simulink model "TEC_Electrothermal_ClosedLoop"  (R2022b)
settings: Solver=ode15s  StartTime=0.0  StopTime=2400  MaxStep=1  RelTol=1e-6  AbsTol=1e-8
model workspace (MAT data in the model file):
  TEC_parameters = [24 0.8 0.012578468121 0.070126334619 4.5 0.02 3 3.6 0.25 0.012 0.2 500]
  switching_mode = 0
libraries: fl_lib x11, nesl_utility x5, ee_lib x1
settings Model: Creator=Greatlovers  LastModifiedBy=Greatlovers

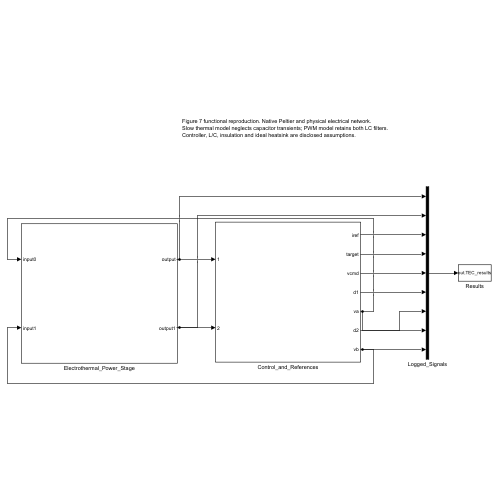
[thumbnail: Simulink's stored preview of the top-level diagram]
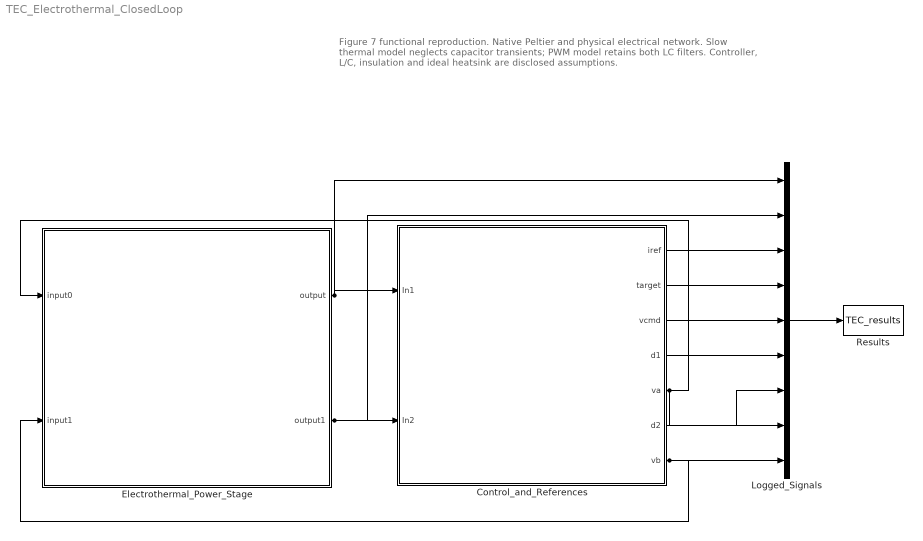
== system TEC_Electrothermal_ClosedLoop ==
  note: Figure 7 functional reproduction. Native Peltier and physical electrical network.
      | Slow thermal model neglects capacitor transients; PWM model retains both LC filters.
      | Controller, L/C, insulation and ideal heatsink are disclosed assumptions.
  Control_and_References : Subsystem
  Electrothermal_Power_Stage : Subsystem
  Logged_Signals : Mux  Inputs=9
  Results : ToWorkspace  VariableName=TEC_results  SaveFormat=Timeseries  SampleTime=-1
  wires:
  Control_and_References/4(d1) -> Logged_Signals/6
  Electrothermal_Power_Stage/1(output) -> Logged_Signals/1, Control_and_References/1(In1)
  Control_and_References/3(vcmd) -> Logged_Signals/5
  Control_and_References/1(iref) -> Logged_Signals/3
  Electrothermal_Power_Stage/2(output1) -> Logged_Signals/2, Control_and_References/2(In2)
  Control_and_References/2(target) -> Logged_Signals/4
  Control_and_References/5(va) -> Electrothermal_Power_Stage/1(input0), Logged_Signals/8
  Control_and_References/6(d2) -> Logged_Signals/7
  Control_and_References/7(vb) -> Electrothermal_Power_Stage/2(input1), Logged_Signals/9
  Logged_Signals/1 -> Results/1

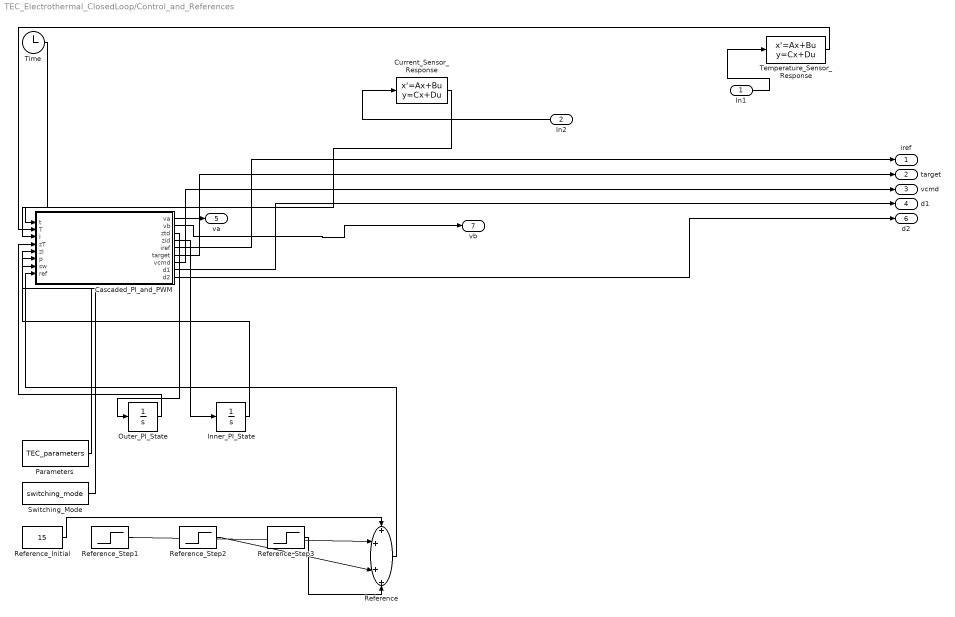
== system TEC_Electrothermal_ClosedLoop/Control_and_References ==
  In1 : Inport
  In2 : Inport  Port=2
  Cascaded_PI_and_PWM : MATLAB Function  TreatAsAtomicUnit=on
  Current_Sensor_Response : StateSpace  A=-1e5  B=1e5  D=0  InitialCondition=0
  Inner_PI_State : Integrator
  Outer_PI_State : Integrator
  Parameters : Constant  Value=TEC_parameters
  Reference : Sum  Inputs=++++
  Reference_Initial : Constant  Value=15
  Reference_Step1 : Step  Time=600  After=40  SampleTime=0
  Reference_Step2 : Step  Time=1200  After=-70  SampleTime=0
  Reference_Step3 : Step  Time=1800  After=110  SampleTime=0
  Switching_Mode : Constant  Value=switching_mode
  Temperature_Sensor_Response : StateSpace  A=-100  B=100  D=0  InitialCondition=298.15
  Time : Clock
  iref : Outport
  target : Outport  Port=2
  vcmd : Outport  Port=3
  d1 : Outport  Port=4
  va : Outport  Port=5
  d2 : Outport  Port=6
  vb : Outport  Port=7
  wires:
  Reference_Step3/1 -> Reference/4
  Reference_Initial/1 -> Reference/1
  Outer_PI_State/1 -> Cascaded_PI_and_PWM/4(zT)
  Cascaded_PI_and_PWM/1(va) -> va/1
  Time/1 -> Cascaded_PI_and_PWM/1(t)
  Reference_Step1/1 -> Reference/2
  Current_Sensor_Response/1 -> Cascaded_PI_and_PWM/3(I)
  Switching_Mode/1 -> Cascaded_PI_and_PWM/7(sw)
  Cascaded_PI_and_PWM/9(d2) -> d2/1
  Reference/1 -> Cascaded_PI_and_PWM/8(ref)
  Temperature_Sensor_Response/1 -> Cascaded_PI_and_PWM/2(T)
  Reference_Step2/1 -> Reference/3
  Cascaded_PI_and_PWM/5(iref) -> iref/1
  Inner_PI_State/1 -> Cascaded_PI_and_PWM/5(zI)
  Parameters/1 -> Cascaded_PI_and_PWM/6(p)
  Cascaded_PI_and_PWM/3(ztd) -> Outer_PI_State/1
  In1/1 -> Temperature_Sensor_Response/1
  Cascaded_PI_and_PWM/4(zid) -> Inner_PI_State/1
  In2/1 -> Current_Sensor_Response/1
  Cascaded_PI_and_PWM/8(d1) -> d1/1
  Cascaded_PI_and_PWM/2(vb) -> vb/1
  Cascaded_PI_and_PWM/7(vcmd) -> vcmd/1
  Cascaded_PI_and_PWM/6(target) -> target/1

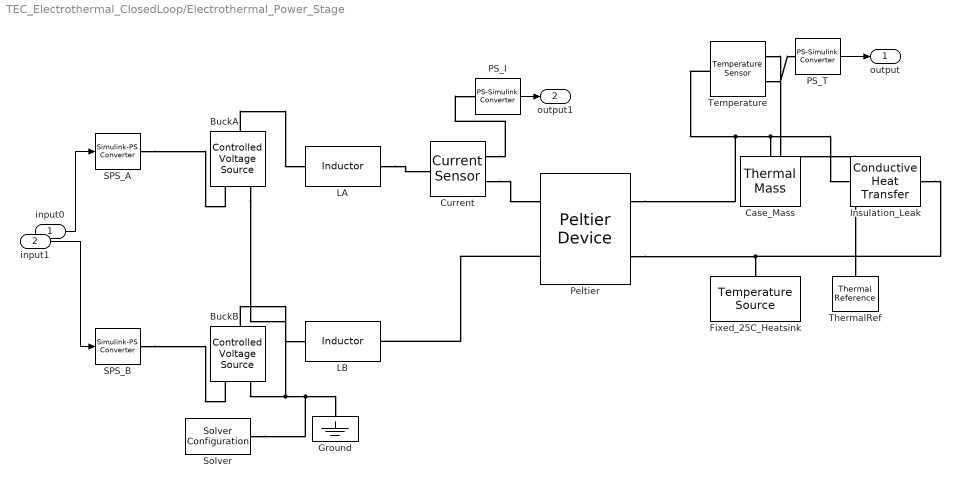
== system TEC_Electrothermal_ClosedLoop/Electrothermal_Power_Stage ==
  input0 : Inport
  input1 : Inport  Port=2
  BuckA : fl_lib/Electrical/Electrical Sources/Controlled Voltage Source
  BuckB : fl_lib/Electrical/Electrical Sources/Controlled Voltage Source
  Case_Mass : fl_lib/Thermal/Thermal Elements/Thermal Mass  mass=0.005 kg  sp_heat=900 J/(K*kg)  num_ports=foundation.enum.numPorts2.one  T_specify=on  T_priority=High  T=298.15 K  T_nominal_specify=off  T_nominal_unit=K  T_nominal_value=1  Q_specify=off  Q_priority=None  Q=0 W  Q_nominal_specify=off  Q_nominal_unit=W  Q_nominal_value=1
  Current : fl_lib/Electrical/Electrical Sensors/Current Sensor
  Fixed_25C_Heatsink : fl_lib/Thermal/Thermal Sources/Temperature Source  temperature=298.15 K
  Ground : fl_lib/Electrical/Electrical Elements/Electrical Reference
  Insulation_Leak : fl_lib/Thermal/Thermal Elements/Conductive Heat Transfer  thermal_type=foundation.enum.ConstantVariableTabulated.Constant  wall_geometry=foundation.enum.ConductionWallGeometry.Planar  area=0.001 m^2  thickness=0.05 m  d_in=0.05 m  d_out=0.1 m  L=1 m  th_cond_min=10 W/(K*m)  th_cond=1 W/(K*m)  th_cond_TLU=[413, 401, 392, 383, 371, 357, 342] W/(K*m)  temp_TLU=[200, 273, 400, 600, 800, 1000, 1200] K  T_specify=off  T_priority=None  T=0 K  T_nominal_specify=off  T_nominal_unit=K  T_nominal_value=1  Q_specify=off  Q_priority=None  Q=0 W  Q_nominal_specify=off  Q_nominal_unit=W  Q_nominal_value=1
  LA : fl_lib/Electrical/Electrical Elements/Inductor  l=220e-6 H  r=0.03 Ohm  g=1e-9 1/Ohm  i_specify=off  i_priority=None  i=0 A  i_nominal_specify=off  i_nominal_unit=A  i_nominal_value=1  v_specify=off  v_priority=None  v=0 V  v_nominal_specify=off  v_nominal_unit=V  v_nominal_value=1  i_L_specify=off  i_L_priority=High  i_L=0 A  i_L_nominal_specify=off  i_L_nominal_unit=A  i_L_nominal_value=1
  LB : fl_lib/Electrical/Electrical Elements/Inductor  l=220e-6 H  r=0.03 Ohm  g=1e-9 1/Ohm  i_specify=off  i_priority=None  i=0 A  i_nominal_specify=off  i_nominal_unit=A  i_nominal_value=1  v_specify=off  v_priority=None  v=0 V  v_nominal_specify=off  v_nominal_unit=V  v_nominal_value=1  i_L_specify=off  i_L_priority=High  i_L=0 A  i_L_nominal_specify=off  i_L_nominal_unit=A  i_L_nominal_value=1
  PS_I : nesl_utility/PS-Simulink Converter  PhysicalDomain=network_engine_domain  SubClassName=ps_output  LeftPortType=input  RightPortType=output  PseudoPeriodic=off  Frequencies=[]  VectorFormat=inherit  Unit=A  AffineConversion=off
  PS_T : nesl_utility/PS-Simulink Converter  PhysicalDomain=network_engine_domain  SubClassName=ps_output  LeftPortType=input  RightPortType=output  PseudoPeriodic=off  Frequencies=[]  VectorFormat=inherit  Unit=K  AffineConversion=off
  Peltier : ee_lib/Sensors & Transducers/Peltier Device  alpha=TEC_parameters(3) V/K  R=TEC_parameters(2) Ohm  K=TEC_parameters(4) W/K
      settings: InternalSimscapePortConfiguration="{\"Bottom\":[],\"Left\":[{\"id\":\"p\",\"label\":\"+\",\"type\":\"foundation.electrical.electrical\"},{\"id\":\"n\",\"label\":\"-\",\"type\":\"foundation.electrical.electrical\"}],\"Right\":[{\"id\":\"A\",\"label\":\"A\",\"type\":\"foundation.thermal.thermal\"},{\"id\":\"B\",\"label\":\"B\",\"type\":\"foundation.thermal.thermal\"}],\"Top\":[]}"
  SPS_A : nesl_utility/Simulink-PS Converter  PhysicalDomain=network_engine_domain  SubClassName=ps_input  LeftPortType=input  RightPortType=output  PseudoPeriodic=off  Frequencies=[]  NoiseDistribution=none  NoiseParameters=[]  Unit=V  AffineConversion=off  FilteringAndDerivatives=zero  SimscapeFilterOrder=1  InputFilterTimeConstant=0.001  UdotUserProvided=0
  SPS_B : nesl_utility/Simulink-PS Converter  PhysicalDomain=network_engine_domain  SubClassName=ps_input  LeftPortType=input  RightPortType=output  PseudoPeriodic=off  Frequencies=[]  NoiseDistribution=none  NoiseParameters=[]  Unit=V  AffineConversion=off  FilteringAndDerivatives=zero  SimscapeFilterOrder=1  InputFilterTimeConstant=0.001  UdotUserProvided=0
  Solver : nesl_utility/Solver Configuration  PhysicalDomain=network_engine_domain  SubClassName=solver  LeftPortType=input  RightPortType=generic  Tones=[]  Harmonics=[]  SimulateNoise=off  Profile=off  UseLocalSampling=off  EnableSwitchedLinearOptims=on  FrequencyDomain=off  UseCCode=off  RelTol=0.001  AbsTol=0.001  MinStep=1e-09  ToWorkspace=off  RevertToSquareIcSolve=off  NumHomotopyIterations=100  PhasorMode=off  PhasorModeNumHarmonics=1  ConsistencySolver=NEWTON_XTOL_AFTER_FTOL  IndexReductionMethod=DerivativeReplacement  DoDC=off  ResidualTolerance=1e-09  ConsistencyTolSource=GLOBAL  ConsistencyAbsTol=0.001  ConsistencyRelTol=0.001  ConsistencyTolFactor=0.001  UseLocalSolver=off  LocalSolverChoice=NE_BACKWARD_EULER_ADVANCER  ResolveIndetEquations=on  FunctionEvalNumThread=1  LocalSolverSampleTime=0.001  DoFixedCost=off  MaxNonlinIter=3  MaxModeIter=2  ComputeImpulses=off  ImpulseIterations=2  LinearAlgebra=auto  LinearAlgebraNumThread=0  EquationFormulation=NE_TIME_EF  DelaysMemoryBudget=1024  AutomaticFiltering=on  FilteringTimeConstant=0.001  PartitionStorageMethod=AS_NEEDED  PartitionMemoryBudget=1024  PartitionMethod=ROBUST
  Temperature : fl_lib/Thermal/Thermal Sensors/Temperature Sensor
  ThermalRef : fl_lib/Thermal/Thermal Elements/Thermal Reference
  output : Outport
  output1 : Outport  Port=2
  wires:
  input0/1 -> SPS_A/1
  PS_I/1 -> output1/1
  PS_T/1 -> output/1
  input1/1 -> SPS_B/1
  connections:
  BuckA/RConn2 -- Ground/LConn1 -- Solver/RConn1 -- BuckB/RConn2
  Current/RConn2 -- Peltier/LConn1
  Peltier/RConn1 -- Case_Mass/LConn1 -- Insulation_Leak/LConn1 -- Temperature/LConn1
  Temperature/RConn2 -- PS_T/LConn1
  BuckA/LConn1 -- LA/LConn1
  BuckB/LConn1 -- LB/LConn1
  SPS_A/RConn1 -- BuckA/RConn1
  Peltier/LConn2 -- LB/RConn1
  Insulation_Leak/RConn1 -- Fixed_25C_Heatsink/LConn1 -- Peltier/RConn2
  Temperature/RConn1 -- ThermalRef/LConn1
  Current/RConn1 -- PS_I/LConn1
  LA/RConn1 -- Current/LConn1
  SPS_B/RConn1 -- BuckB/RConn1

== matlab function TEC_Electrothermal_ClosedLoop/Control_and_References/Cascaded_PI_and_PWM ==
  data: t input; va output; T input; I input; zT input; zI input; p input; sw input; ref input; vb output; ztd output; zid output; iref output; target output; vcmd output; d1 output; d2 output
function [va,vb,ztd,zid,iref,target,vcmd,d1,d2]=control(t,T,I,zT,zI,p,sw,ref)
if sw>0.5
 target=25;iref=ref;ztd=0;
else
 target=ref;
errT=T-273.15-target; iraw=p(9)*errT+zT;iref=min(p(7),max(-p(7),iraw));ztd=p(10)*errT+0.3*(iref-iraw);
end
errI=iref-I;vraw=(p(2)+0.06)*iref+p(3)*(298.15-T)+p(11)*errI+zI;vcmd=min(p(8),max(-p(8),vraw));zid=p(12)*errI+100*(vcmd-vraw);
d1=0.5+vcmd/(2*p(1));d2=0.5-vcmd/(2*p(1));
if sw>0.5
 carrier=mod(t*20000,1);va=p(1)*double(carrier<d1);vb=p(1)*double(carrier<d2);
else
 va=p(1)*d1;vb=p(1)*d2;
end
end
